simulink model "QD2_MissionCtrl_Dual_MPC"  (R2022b)
settings: Solver=ode2  StartTime=0.0  StopTime=inf  FixedStep=0.001  RelTol=1e-3  EnableMultiTasking=on
PreLoadFcn:
  | % Rutas: simulink_qdrone2 (qd2_cargar_config), lib (qd2_*.m) y la carpeta
  | % del modelo (QD2_Mission_Lib.slx de la misma versión de MATLAB).
  | qd2_d = fileparts(get_param(bdroot, 'FileName')); qd2_r = qd2_d;
  | while ~isempty(qd2_r) && ~exist(fullfile(qd2_r, 'qd2_cargar_config.m'), 'file')
  |     qd2_p = fileparts(qd2_r); if strcmp(qd2_p, qd2_r), qd2_r = ''; else, qd2_r = qd2_p; end
  | end
  | if ~isempty(qd2_r), addpath(fullfile(qd2_r, 'lib')); addpath(qd2_r); end
  | if exist(fullfile(qd2_d, 'QD2_Mission_Lib.slx'), 'file'), addpath(qd2_d); end
  | clear qd2_d qd2_r qd2_p
PostLoadFcn:
  | try, qd2_cargar_config(); catch qd2_e, warning(qd2_e.message); end
InitFcn:
  | qd2_cargar_config(bdroot);
undefined symbols (not defined in the file): _MissionCtrl, _MissionDual, datetime, Host, localhost, log_, m, qc_get_step_size, QD2CFG, QD2P, saved_data
libraries: quarc_library x43, QD2_Mission_Lib x12, simulink x11
(part 1 of 2)
Description:
  | Modelo de tierra para 2 QDrone 2 (versión MPC). Copia extendida de QD2_MissionCtrl_NoJoystick_2021a del Equipo2, generada por simulink_qdrone2/construir_modelos.m. Contrato: docs/ARQUITECTURA.md.
settings Model: SimulationMode=external  ExtModeTrigDuration=10000  Creator=Admin  LastModifiedBy=ezequ
settings SolverCC: AlgebraicLoopSolver=TrustRegion  PositivePriorityOrder=on
settings DataIOCC: ReturnWorkspaceOutputs=off
settings OptimizationCC: ReuseModelBlockBuffer=on
settings DebuggingCC: UnconnectedInputMsg=warning  UnconnectedOutputMsg=warning  UnconnectedLineMsg=warning  SFUnexpectedBacktrackingDiag=warning  SFNoUnconditionalDefaultTransitionDiag=warning  SFExecutionAtInitializationDiag=none  ArithmeticOperatorsInVariantConditions=warning
settings ModelReferenceCC: EnableRefExpFcnMdlSchedulingChecks=on
settings SFSimCC: SimUseLocalCustomCode=off  CustomCodeUndefinedFunction=UseInterfaceOnly
settings RTWCC: Description=QUARC Win64 Target Using Toolchain  SystemTargetFile=quarc_win64.tlc  TemplateMakefile=quarc_default_tmf  RTWUseLocalCustomCode=off  Toolchain=QUARC win64 | nmake (64-bit Windows)  BuildConfiguration=Faster Runs  DLArmComputeVersion=19.05
settings CodeAppCC: StateflowObjectComments=on
settings STFCustomTargetCC: ConcurrentExecutionCompliant=on  GRTInterface=on  UseToolchainInfoCompliant=on  SystemTargetFile=quarc_win64.tlc
settings GRTTargetCC: TargetLangStandard=C89/C90 (ANSI)  ParMdlRefBuildCompliant=off  CompOptLevelCompliant=off  CombineOutputUpdateFcns=off  MatFileLogging=off  CPPClassGenCompliant=off  GRTInterface=on  ExtMode=on  ExtModeMexFile=quarc_comm  ExtModeMexArgs='-w -d %d -uri %u -URI_Host tcpip://localhost:18001 -URI_Host2 tcpip://localhost:18002'
settings ConfigComp: CovMetricSettings=dw  CovSaveCumulativeToWorkspaceVar=on  CovSaveSingleToWorkspaceVar=on  CovExternalEMLEnable=off  CovBoundaryAbsTol=1.0e-5

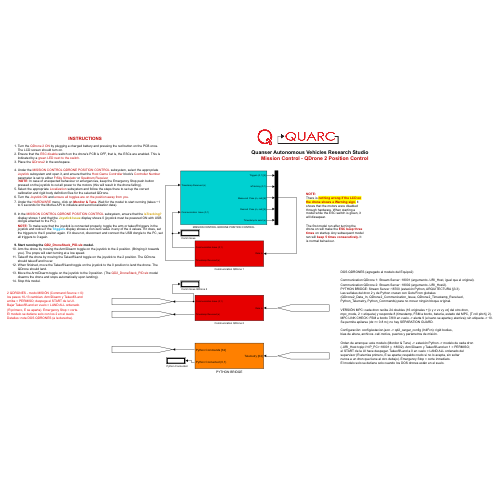
[thumbnail: Simulink's stored preview of the top-level diagram]
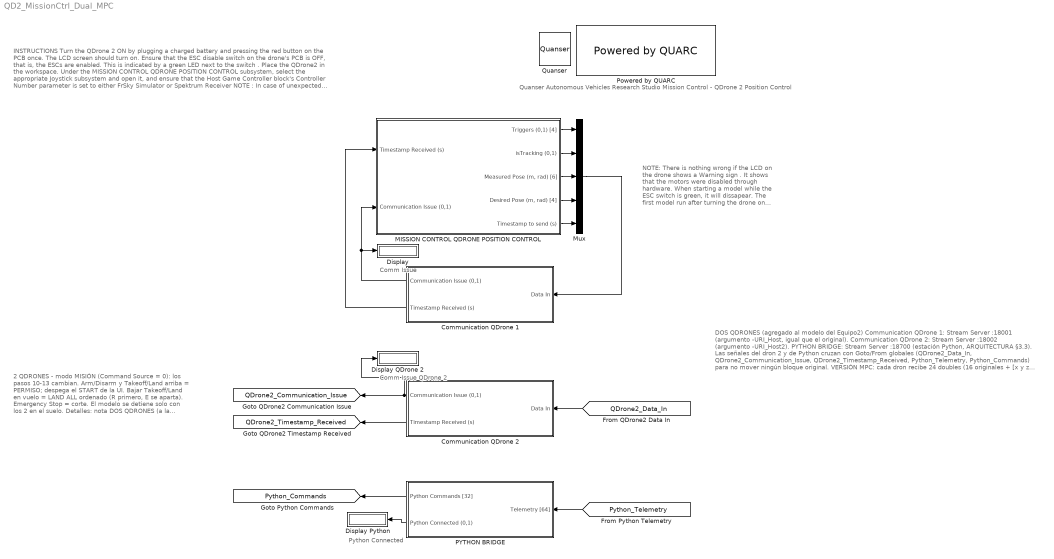
== system QD2_MissionCtrl_Dual_MPC ==
  note: Quanser Autonomous Vehicles Research Studio
      | Mission Control - QDrone 2 Position Control
  note: Comm Issue
  note: INSTRUCTIONS
      |
      | Turn the QDrone 2 ON by plugging a charged battery and pressing the red button on the PCB once. The LCD screen should turn on.
      | Ensure that the ESC disable switch on the drone's PCB is OFF, that is, the ESCs are enabled. This is indicated by a green LED next to the switch .
      | Place the QDrone2 in the workspace.
      |
      | Under the MISSION CONTROL QDRONE POSITION CONTROL subsystem, select the appropriate Joystick subsystem and open it, and ensure that the Host Game Controller block's Controller Number parameter is set to either FrSky Simulator or Spektrum Receiver
      | NOTE : In case of unexpected behaviour or emergencies, keep the Emergency Stop push button pressed on the joystick to cut all power to the motors (this will result in the drone falling).
      | Select the appropriate Localization subsystem and follow the steps there to set up the correct calibration and rigid body definition files for the selected QDrone.
      | Turn the Joystick ON and ensure all toggles are on the position away from you .
      | Under the HARDWARE menu, click on Monitor & Tune . Wait for the model to start running (takes ~1 to 5 seconds for the Motive API to initialize and send localization data).
      |
      | In the MISSION CONTROL QDRONE POSITION CONTROL subsystem, ensure that the isTracking? display shows 1 and that the Joystick Issue display shows 0 (joystick must be powered ON with USB dongle attached to the PC).
      | NOTE: To make sure that the joystick is connected properly, toggle the arm or takeoff triggers in the joystick and notice if the Triggers display shows a non zero value in any of the 4 values. If it does, set the triggers to the 0 positon again. If it does not, disconnect and connect the USB dongle to the PC, set all triggers to 0 again.
      |
      | Start running the QD2_DroneStack_PID.slx model.
      | Arm the drone by moving the Arm/Disarm toggle on the joystick to the 2 position. (Bringing it towards you). The props will start turning at a low speed.
      | Takeoff the drone by moving the Takeoff/Land toggle on the joystick to the 2 position. The QDrone should takeoff and hover.
      | When finished, move the Takeoff/Land toggle on the joystick to the 0 position to land the drone. The QDrone should land.
      | Move the Arm/Disarm toggle on the joystick to the 0 position. (The QD2_DroneStack_PID.sl x model disarms the drone and stops automatically upon landing).
      | Stop this model.
  note: NOTE:
      | There is nothing wrong if the LCD on the drone shows a Warning sign . It shows that the motors were disabled through hardware. When starting a model while the ESC switch is green, it will dissapear.
      |
      | The first model run after turning the drone on will make the ESC beep three times on startup. Any subsequent model ran will beep 5 times consecutively. It is normal behaviour.
  note: Comm Issue QDrone 2
  note: Python Connected
  note: DOS QDRONES (agregado al modelo del Equipo2)
      |
      | Communication QDrone 1: Stream Server :18001 (argumento -URI_Host, igual que el original).
      | Communication QDrone 2: Stream Server :18002 (argumento -URI_Host2).
      | PYTHON BRIDGE: Stream Server :18700 (estación Python, ARQUITECTURA §3.3).
      | Las señales del dron 2 y de Python cruzan con Goto/From globales
      | (QDrone2_Data_In, QDrone2_Communication_Issue, QDrone2_Timestamp_Received,
      | Python_Telemetry, Python_Commands) para no mover ningún bloque original.
      |
      | VERSIÓN MPC: cada dron recibe 24 doubles (16 originales + [x y z vx vy vz] del otro dron,
      | mpc_mode, 2 = etiqueta) y responde 8 (timestamp, FSM a bordo, batería, estado del MPC, [T roll pitch], 2).
      | MPC LINK CHECK: FSM a bordo 7/8/9 en vuelo -> alerta 9 (el sano se aparta y aterriza); sin etiqueta -> 10.
      | Se permite apilarse (dz >= 0.8 m); no hay SEPARATION GUARD.
      |
      | Configuración: config/estacion.json -> qd2_cargar_config (InitFcn): rigid bodies,
      | bias de altura, archivos .cal/.motive, puertos y parámetros de misión.
      |
      | Orden de arranque: este modelo (Monitor & Tune) -> estación Python -> modelo de cada dron
      | (-URI_Host tcpip://<IP_PC>:18001 y :18002). Arm/Disarm y Takeoff/Land en 1 = PERMISO;
      | el START de la UI hace despegar. Takeoff/Land a 0 en vuelo = LAND ALL ordenado del
      | supervisor (R aterriza primero, E se aparta; respaldo crudo si no lo acepta, sin soltar
      | nunca a un dron que tiene al otro debajo). Emergency Stop = corte inmediato.
      | El modelo solo se detiene solo cuando los DOS drones están en el suelo.
  note: 2 QDRONES - modo MISIÓN (Command Source = 0):
      | los pasos 10-13 cambian. Arm/Disarm y Takeoff/Land
      | arriba = PERMISO; despega el START de la UI.
      | Bajar Takeoff/Land en vuelo = LAND ALL ordenado
      | (R primero, E se aparta). Emergency Stop = corte.
      | El modelo se detiene solo con los 2 en el suelo.
      | Detalles: nota DOS QDRONES (a la derecha).
  Communication QDrone 1 : Subsystem
  Communication QDrone 2 : Subsystem
  Display : Display
  Display Python : Display
  Display QDrone 2 : Display
  MISSION CONTROL QDRONE POSITION CONTROL : Subsystem
  Mux : Mux  Inputs=5
  PYTHON BRIDGE : Subsystem
  Powered by QUARC : quarc_library/Logos/Powered by QUARC
  Quanser : quarc_library/Logos/Quanser
  tag scope: Python_Commands=global, QDrone2_Communication_Issue=global, QDrone2_Timestamp_Received=global
  wires:
  Communication QDrone 1/2(Timestamp Received (s)) -> MISSION CONTROL QDRONE POSITION CONTROL/1(Timestamp Received (s))
  MISSION CONTROL QDRONE POSITION CONTROL/5(Timestamp to send (s)) -> Mux/5
  Mux/1 -> Communication QDrone 1/1(Data In)
  Communication QDrone 1/1(Communication Issue (0,1)) -> MISSION CONTROL QDRONE POSITION CONTROL/2(Communication Issue (0,1)), Display/1
  MISSION CONTROL QDRONE POSITION CONTROL/3("Measured Pose (m, rad) [6]") -> Mux/3
  MISSION CONTROL QDRONE POSITION CONTROL/4("Desired Pose (m, rad) [4]") -> Mux/4
  MISSION CONTROL QDRONE POSITION CONTROL/1(Triggers (0,1) [4]) -> Mux/1
  MISSION CONTROL QDRONE POSITION CONTROL/2(isTracking (0,1)) -> Mux/2
  [QDrone2_Data_In] -> Communication QDrone 2/1(Data In)
  Communication QDrone 2/1(Communication Issue (0,1)) -> [QDrone2_Communication_Issue], Display QDrone 2/1
  Communication QDrone 2/2(Timestamp Received (s)) -> [QDrone2_Timestamp_Received]
  [Python_Telemetry] -> PYTHON BRIDGE/1(Telemetry [64])
  PYTHON BRIDGE/1(Python Commands [32]) -> [Python_Commands]
  PYTHON BRIDGE/2(Python Connected (0,1)) -> Display Python/1

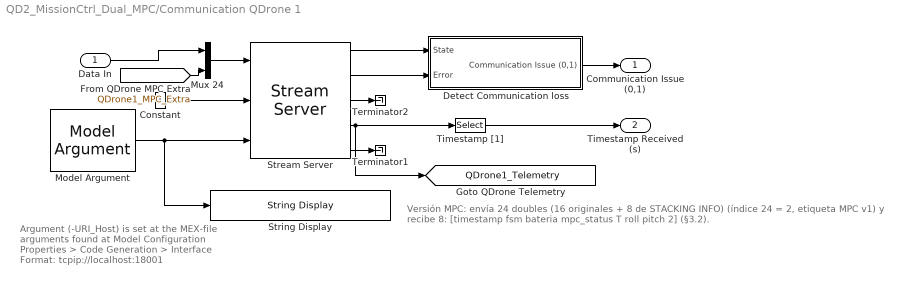
== system QD2_MissionCtrl_Dual_MPC/Communication QDrone 1 ==
  note: Argument (-URI_Host) is set at the MEX-file arguments
      | found at Model Configuration Properties > Code Generation > Interface
      |
      | Format:
      | tcpip://localhost:18001
  note: Versión MPC: envía 24 doubles (16 originales + 8 de STACKING INFO)
      | (índice 24 = 2, etiqueta MPC v1) y recibe 8: [timestamp fsm bateria mpc_status T roll pitch 2] (§3.2).
  Data In : Inport
  Constant : Constant
  Detect Communication loss : Subsystem
  Model Argument : quarc_library/Sources/Signals/Model Argument  argument_name=URI_Host  has_value=on  data_type_mode=Specify via dialog  data_type=char  max_length=80  default_value=0  variable_size=off
      settings: AttributesFormatString=(-%<argument_name>)  SourceProductName=QUARC Targets
  Mux 24 : Mux  Inputs=2
  Stream Server : quarc_library/Communications/Basic/Stream Server  uri_source=External input port  uri=tcpip://localhost:18877  send_buffer_size=1460  receive_buffer_size=1460  byte_order=little endian (Intel - LSB first)  optimization=Minimum latency  send_options=Send most recent data  receive_options=Receive most recent data  default_value=[0; NaN(7,1)]  sample_time=qc_get_step_size  active=off  implementation=Use blocking I/O in a separate thread  send_fifo_size=1000  receive_fifo_size=1000  send_priority=0  receive_priority=0  send_dimensions=off  receive_dimensions=off  max_dimensions=-1  data_type=Inherited via back propagation  type_expr=BusObject
  "String Display " : quarc_library/Strings/String Display  alignment=center  display_mode=Single line  sample_time=-1  use_new=off
      settings: SourceProductName=QUARC Targets
  Terminator1 : Terminator
  Terminator2 : Terminator
  Timestamp [1] : Selector  InputPortWidth=8  IndexOptions=Index vector (dialog)  Indices=1  OutputSizes=1
  Communication Issue (0,1) : Outport  VectorParamsAs1DForOutWhenUnconnected=off
  Timestamp Received (s) : Outport  Port=2  VectorParamsAs1DForOutWhenUnconnected=off
  tag scope: QDrone1_Telemetry=global
  wires:
  Constant/1 -> Stream Server/2
  Stream Server/3 -> Terminator2/1
  Stream Server/5 -> Terminator1/1
  Model Argument/1 -> "String Display "/1, Stream Server/3
  Stream Server/1 -> Detect Communication loss/1(State)
  Stream Server/2 -> Detect Communication loss/2(Error)
  Detect Communication loss/1(Communication Issue (0,1)) -> Communication Issue (0,1)/1
  Data In/1 -> Mux 24/1
  [QDrone1_MPC_Extra] -> Mux 24/2
  Mux 24/1 -> Stream Server/1
  Stream Server/4 -> Timestamp [1]/1, [QDrone1_Telemetry]
  Timestamp [1]/1 -> Timestamp Received (s)/1

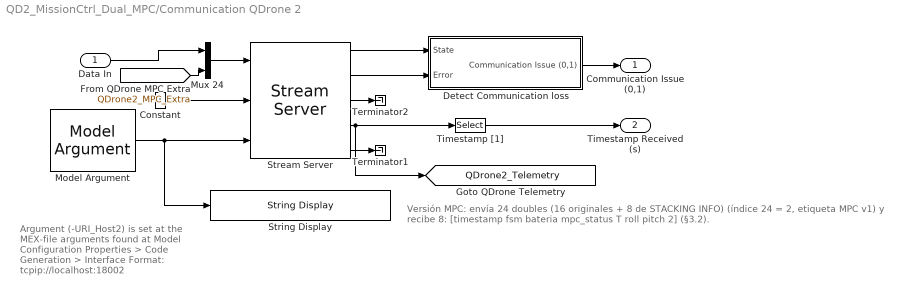
== system QD2_MissionCtrl_Dual_MPC/Communication QDrone 2 ==
  note: Versión MPC: envía 24 doubles (16 originales + 8 de STACKING INFO)
      | (índice 24 = 2, etiqueta MPC v1) y recibe 8: [timestamp fsm bateria mpc_status T roll pitch 2] (§3.2).
  note: Argument (-URI_Host2) is set at the MEX-file arguments
      | found at Model Configuration Properties > Code Generation > Interface
      |
      | Format:
      | tcpip://localhost:18002
  Data In : Inport
  Constant : Constant
  Detect Communication loss : Subsystem
  Model Argument : quarc_library/Sources/Signals/Model Argument  argument_name=URI_Host2  has_value=on  data_type_mode=Specify via dialog  data_type=char  max_length=80  default_value=0  variable_size=off
      settings: AttributesFormatString=(-%<argument_name>)  SourceProductName=QUARC Targets
  Mux 24 : Mux  Inputs=2
  Stream Server : quarc_library/Communications/Basic/Stream Server  uri_source=External input port  uri=tcpip://localhost:18877  send_buffer_size=1460  receive_buffer_size=1460  byte_order=little endian (Intel - LSB first)  optimization=Minimum latency  send_options=Send most recent data  receive_options=Receive most recent data  default_value=[0; NaN(7,1)]  sample_time=qc_get_step_size  active=off  implementation=Use blocking I/O in a separate thread  send_fifo_size=1000  receive_fifo_size=1000  send_priority=0  receive_priority=0  send_dimensions=off  receive_dimensions=off  max_dimensions=-1  data_type=Inherited via back propagation  type_expr=BusObject
  "String Display " : quarc_library/Strings/String Display  alignment=center  display_mode=Single line  sample_time=-1  use_new=off
      settings: SourceProductName=QUARC Targets
  Terminator1 : Terminator
  Terminator2 : Terminator
  Timestamp [1] : Selector  InputPortWidth=8  IndexOptions=Index vector (dialog)  Indices=1  OutputSizes=1
  Communication Issue (0,1) : Outport  VectorParamsAs1DForOutWhenUnconnected=off
  Timestamp Received (s) : Outport  Port=2  VectorParamsAs1DForOutWhenUnconnected=off
  tag scope: QDrone2_Telemetry=global
  wires:
  Timestamp [1]/1 -> Timestamp Received (s)/1
  Stream Server/4 -> [QDrone2_Telemetry], Timestamp [1]/1
  Mux 24/1 -> Stream Server/1
  [QDrone2_MPC_Extra] -> Mux 24/2
  Data In/1 -> Mux 24/1
  Detect Communication loss/1(Communication Issue (0,1)) -> Communication Issue (0,1)/1
  Stream Server/2 -> Detect Communication loss/2(Error)
  Stream Server/1 -> Detect Communication loss/1(State)
  Model Argument/1 -> Stream Server/3, "String Display "/1
  Stream Server/5 -> Terminator1/1
  Stream Server/3 -> Terminator2/1
  Constant/1 -> Stream Server/2

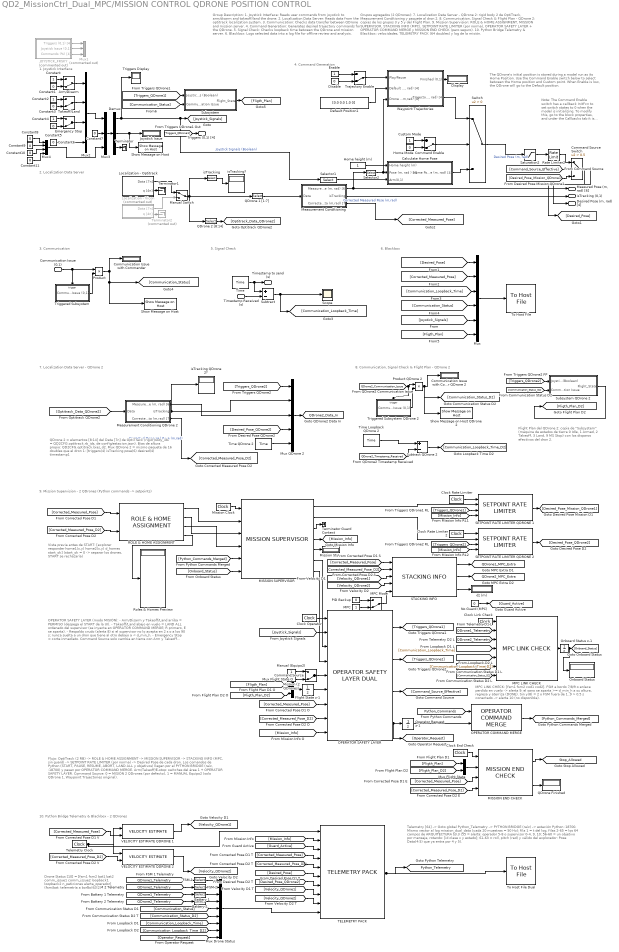
== system QD2_MissionCtrl_Dual_MPC/MISSION CONTROL QDRONE POSITION CONTROL ==
  note: 5. Signal Check
  note: 6. Blackbox
  note: 3. Communication
  note: 2. Localization Data Server
  note: 1. Joystick Interface
  note: 4. Command Generation
  note: Group Description:
      |
      | 1. Joystick Interface: Reads user commands from joystick to arm/disarm and takeoff/land the drone.
      | 2. Localization Data Server: Reads data from the optitrack localization system.
      | 3. Communication: Checks data transfer between QDrone and mission server.
      | 4. Command Generation: Generates desired trajectory commands for the QDrone.
      | 5. Signal Check: Checks loopback time between the QDrone and mission server.
      | 6. Blackbox: Logs selected data into a log file for offline review and analysis.
  note: The QDrone's initial position is stored during a model run as its Home Position.
      | Use the Command Enable switch below to select between the Home position and Custom point. When Enable is low, the QDrone will go to the Default position.
  note: Note:
      | The Command Enable switch has a callback InitFcn to set switch states to 0 when the model is initializing. To modify this, go to the block properties, and under the Callbacks tab it is set in the InitFcn.
  note: 7. Localization Data Server - QDrone 2
  note: 8. Communication, Signal Check & Flight Plan - QDrone 2
  note: 9. Mission Supervision - 2 QDrones (Python commands -> setpoints)
  note: 10. Python Bridge Telemetry & Blackbox - 2 QDrones
  note: Grupos agregados (2 QDrones):
      |
      | 7. Localization Data Server - QDrone 2: rigid body 2 de OptiTrack, Measurement Conditioning y paquete al dron 2.
      | 8. Communication, Signal Check & Flight Plan - QDrone 2: copias de los grupos 3 y 5 y del Flight Plan.
      | 9. Mission Supervision: ROLE & HOME ASSIGNMENT, MISSION SUPERVISOR, STACKING INFO (MPC),
      |    SETPOINT RATE LIMITER (por norma), OPERATOR SAFETY LAYER + OPERATOR COMMAND MERGE y MISSION END CHECK (paro seguro).
      | 10. Python Bridge Telemetry & Blackbox: velocidades, TELEMETRY PACK (64 doubles) y log de la misión.
  note: QDrone 2 = elementos [8:14] del Data [7n] de OptiTrack
      | (rigid_body_ids = QD2CFG.optitrack.rb_ids, de config/estacion.json).
      | Bias de altura propio: QD2CFG.optitrack.bias_d2.
      | Mux QDrone 2 = mismo paquete de 16 doubles que el dron 1:
      | [triggers(4) isTracking pose(6) desired(4) timestamp].
  note: Flight Plan del QDrone 2: copia de "Subsystem"
      | (máquina de estados de tierra 0 Idle, 1 Armed,
      | 2 Takeoff, 3 Land, 9 MS Stop) con los disparos
      | efectivos del dron 2.
  note: Vista previa antes de START:
      | [explorer responder home1(x,y) home2(x,y)
      |  d_homes start_ok]  (start_ok = 0 ->
      |  separar los drones, START se rechazaría)
  note: OPERATOR SAFETY LAYER (modo MISIÓN):
      | - Arm/Disarm y Takeoff/Land arriba = PERMISO (despega el START de la UI).
      | - Takeoff/Land abajo en vuelo = LAND ALL ordenado del supervisor
      |   (se inyecta en OPERATOR COMMAND MERGE; R primero, E se aparta).
      | - Respaldo crudo (alerta 8) si el supervisor no lo acepta en 2 s o a los
      |   90 s; nunca suelta a un dron que tiene al otro debajo a < d_min_h.
      | - Emergency Stop = corte inmediato. Command Source solo cambia en
      |   tierra con Arm y Takeoff abajo.
  note: MPC LINK CHECK: [fsm1 fsm2 cod1 cod2]. FSM a bordo 7/8/9 o enlace perdido en vuelo
      | -> alerta 9: el sano se aparta >= d_min_h a su altura, regresa y aterriza (DONE).
      | Sin y(8) = 2 o FSM fuera de 1..9 > 0.5 s conectado -> alerta 10 (no disponible).
  note: Flujo: OptiTrack (2 RB) -> ROLE & HOME ASSIGNMENT -> MISSION SUPERVISOR -> STACKING INFO (MPC, sin guard)
      | -> SETPOINT RATE LIMITER (por norma) -> Desired Pose de cada dron. Los comandos de Python (START, PAUSE, RESUME,
      | ABORT, LAND ALL y objetivos) llegan por el PYTHON BRIDGE (raíz, :18700) y pasan por OPERATOR COMMAND MERGE.
      | Arm/Takeoff/E-stop: switches del área 1 + OPERATOR SAFETY LAYER. Command Source: 0 = MISIÓN 2 QDrones (por defecto),
      | 1 = MANUAL Equipo2 (solo QDrone 1, Waypoint Trajectories original).
  note: Drone Status [10] = [fsm1 fsm2 bat1 bat2
      | comm_issue1 comm_issue2 loopback1
      | loopback2 n_peticiones alerta_operador]
      | (fsm/bat: telemetría a bordo, §3.2)
  note: Telemetry [64] -> Goto global Python_Telemetry -> PYTHON BRIDGE (raíz) -> estación Python :18700.
      | Mismo vector al log mission_dual_data (cada 20 muestras = 50 Hz): fila 1 = t del log,
      | filas 2-65 = los 64 campos de ARQUITECTURA §3.3 (55 = alerta: operador 5-8 o supervisor 0-4, 9, 10;
      | 56-60 = un objetivo por mensaje, rotando: [id clase x y estado];
      | 61-63 = roll, pitch (rad) y válido del explorador: Pose Data(4:5) que ya entra por 4 y 5).
  Timestamp Received (s) : Inport
  Communication Issue (0,1) : Inport  Port=2
  Arm/Disarm : ManualSwitch  InitFcn=set_param(gcb,'sw','0')  CurrentSetting=0
  Battery 1 : Selector  InputPortWidth=8  IndexOptions=Index vector (dialog)  Indices=3  OutputSizes=1
  Battery 2 : Selector  InputPortWidth=8  IndexOptions=Index vector (dialog)  Indices=3  OutputSizes=1
  Calculate Home Pose : Subsystem
  Clock End Check : DigitalClock  SampleTime=qc_get_step_size
  Clock Link Check : DigitalClock  SampleTime=qc_get_step_size
  Clock Operator : DigitalClock  SampleTime=qc_get_step_size
  Clock Rate Limiter : DigitalClock  SampleTime=qc_get_step_size
  Clock Rate Limiter 2 : DigitalClock  SampleTime=qc_get_step_size
  Command Enable : ManualSwitch  InitFcn=set_param(gcb,'sw','0')  CurrentSetting=0
  Command Source : ManualSwitch  InitFcn=set_param(gcb,'sw','0')  CurrentSetting=0
  Command Source Switch : Switch  Criteria=u2 > Threshold  Threshold=0.5  SaturateOnIntegerOverflow=off  InputSameDT=off
  Communication Issue with Commander : Display
  Communication Issue with Commander QDrone 2 : Display
  Constant : Constant
  Constant{1,3,5..11} (9 alike) : Constant  Value=0
  Constant2 : Constant
  Constant4 : Constant
  Custom Mode : Constant
  Default Position1 : Constant  Value=[0.0 0.0 1.0 0]
  Demux : Demux  Outputs=[4 1 4]
  Disable : Constant  Value=0
  Display : Display
  Emergency Stop : ManualSwitch  InitFcn=set_param(gcb,'sw','0')  CurrentSetting=0
  Enable : Constant
  FSM 1 : Selector  InputPortWidth=8  IndexOptions=Index vector (dialog)  Indices=2  OutputSizes=1
  FSM 2 : Selector  InputPortWidth=8  IndexOptions=Index vector (dialog)  Indices=2  OutputSizes=1
  Flight State z-1 : UnitDelay  InitialCondition=[0; 0]  SampleTime=qc_get_step_size  HasFrameUpgradeWarning=on
  Home Mode : Constant  Value=0
  Home height (m) : Constant
  JOYSTICK_FRSKY : Subsystem  Commented=on
      mask Display: image('$imagefile'); % Use "Edit Image" on toolstrip to change.
  Joystick Issue : Display
  Localization - Optitrack : Subsystem
      mask Display: image('$imagefile'); % Use "Edit Image" on toolstrip to change.
  Localization - Vicon : Subsystem  Commented=on
      mask Display: image('$imagefile'); % Use "Edit Image" on toolstrip to change.
  MISSION END CHECK : QD2_Mission_Lib/MISSION END CHECK  Ts=qc_get_step_size
  MISSION SUPERVISOR : QD2_Mission_Lib/MISSION SUPERVISOR  P=QD2P  version=2  Ts=qc_get_step_size
  MPC : Constant
  MPC LINK CHECK : QD2_Mission_Lib/MPC LINK CHECK  P=QD2P  version=2  Ts=qc_get_step_size
  MPC Mode : ManualSwitch  InitFcn=set_param(gcb,'sw','0')  CurrentSetting=0
  Manual (Equipo2) : Constant
  Manual Switch : ManualSwitch
  Measurement Conditioning : Subsystem
  Measurement Conditioning QDrone 2 : Subsystem
  Mission (2 QDrones) : Constant  Value=0
  Mission Clock : DigitalClock  SampleTime=qc_get_step_size
  Mission State : Display
  Mux : Mux  Inputs=6
  Mux Drone Status : Mux  Inputs=[1 1 1 1 1 1 1 1 2]
  Mux Flight State : Mux  Inputs=2
  Mux Flight State O : Mux  Inputs=2
  Mux QDrone 2 : Mux  Inputs=5
  Mux1 : Mux  Commented=on  Inputs=[4 1 4]
  Mux2 : Mux
  Mux3 : Mux  Inputs=3
  Mux4 : Mux
  No Guard (MPC) : Constant  Value=0
  OPERATOR COMMAND MERGE : QD2_Mission_Lib/OPERATOR COMMAND MERGE  Ts=qc_get_step_size
  OPERATOR SAFETY LAYER : QD2_Mission_Lib/OPERATOR SAFETY LAYER DUAL  P=QD2P  Ts=qc_get_step_size
  Onboard Status : Display
  Onboard Status z-1 : UnitDelay  InitialCondition=[0; 0; 0; 0]  SampleTime=qc_get_step_size  HasFrameUpgradeWarning=on
  Operator Request z-1 : UnitDelay  InitialCondition=[0; 0]  SampleTime=qc_get_step_size  HasFrameUpgradeWarning=on
  PID Backup : Constant  Value=0
  Product : Product
  Product QDrone 2 : Product
  QDrone 1 [1:7] : Selector  InputPortWidth=14  IndexOptions=Index vector (dialog)  Indices=1:7  OutputSizes=1
  QDrone 2 [8:14] : Selector  InputPortWidth=14  IndexOptions=Index vector (dialog)  Indices=8:14  OutputSizes=1
  QDrone Finished : Display
  ROLE & HOME ASSIGNMENT : QD2_Mission_Lib/ROLE & HOME ASSIGNMENT  P=QD2P  version=2  Ts=qc_get_step_size
  Rate Limiter2 : RateLimiter  RisingSlewLimit=[1/3 1/3 1/6 pi/6]  FallingSlewLimit=[-1/3 -1/3 -1/6 -pi/6]  SampleTimeMode=inherited
  Roles & Homes Preview : Display
  SETPOINT RATE LIMITER QDRONE 1 : QD2_Mission_Lib/SETPOINT RATE LIMITER  P=QD2P  dron=1  Ts=qc_get_step_size
  SETPOINT RATE LIMITER QDRONE 2 : QD2_Mission_Lib/SETPOINT RATE LIMITER  P=QD2P  dron=2  Ts=qc_get_step_size
  STACKING INFO : QD2_Mission_Lib/STACKING INFO  Ts=qc_get_step_size
  Saturation2 : Saturate  UpperLimit=[1.5 1.5 1.5 3*pi]  LowerLimit=[-1.5 -1.5 0 -3*pi]
  Scope : Scope
  Selector1 : Selector  InputPortWidth=4  IndexOptions=Index vector (dialog)  Indices=[1]  OutputSizes=1
  Selector2 : Selector  InputPortWidth=6  IndexOptions=Index vector (dialog)  Indices=[1:3,6]  OutputSizes=1
  Show Message on Host : quarc_library/Sinks/Error Handling/Show Message on Host  message_type=Fixed error message  message_icon=Warning  message=Mission Control: No communication with QDrone
      settings: AttributesFormatString="\"%<message>\""  SourceProductName=QUARC Targets
  "Show Message on Host " : quarc_library/Sinks/Error Handling/Show Message on Host  message_type=Fixed error message  message_icon=Warning  message=Mission Control: Joystick Disconnected
      settings: AttributesFormatString="\"%<message>\""  SourceProductName=QUARC Targets
  Show Message on Host QDrone 2 : quarc_library/Sinks/Error Handling/Show Message on Host  message_type=Fixed error message  message_icon=Warning  message=Mission Control: No communication with QDrone 2
      settings: AttributesFormatString="\"%<message>\""  SourceProductName=QUARC Targets
  Subsystem : Subsystem
  Subsystem QDrone 2 : Subsystem
  Subtract : Sum  Inputs=+-
  Subtract QDrone 2 : Sum  Inputs=+-
  Switch : Switch  Criteria=u2 > Threshold  SaturateOnIntegerOverflow=off  InputSameDT=off
  TELEMETRY PACK : QD2_Mission_Lib/TELEMETRY PACK  version=2  Ts=qc_get_step_size
  Takeoff/Land : ManualSwitch  InitFcn=set_param(gcb,'sw','0')  CurrentSetting=0
  Telemetry Clock : DigitalClock  SampleTime=qc_get_step_size
  Terminator : Terminator
  Terminator Guard Context : Terminator
  Terminator1 : Terminator
  Terminator2 : Terminator  Commented=on
  Time : quarc_library/Sources/Time/Time  time_source=Wall clock  sample_time=qc_get_step_size
  Time Loopback QDrone 2 : quarc_library/Sources/Time/Time  time_source=Wall clock  sample_time=qc_get_step_size
  Time QDrone 2 : quarc_library/Sources/Time/Time  time_source=Wall clock  sample_time=qc_get_step_size
  To Host File : quarc_library/Sinks/To Host/To Host File  source=Specify via dialog (do not evaluate)  file_name=saved_data/%m/log_%{regexprep(char(datetime),' ','_')}_MissionCtrl.mat  variable_name=mission_server_data  decimation=1  sample_time=-1  file_format=MAT-file v.5  options=No header or footer  append=off  final_file_name=saved_data/QD2_MissionCtrl_Dual_MPC/log_22-Nov-2026_19-01-13_MissionCtrl.mat  encoding=Default  bitrate=2000000
  To Host File Dual : quarc_library/Sinks/To Host/To Host File  source=Specify via dialog (do not evaluate)  file_name=saved_data/%m/log_%{regexprep(char(datetime),' ','_')}_MissionDual.mat  variable_name=mission_dual_data  decimation=20  sample_time=-1  file_format=MAT-file v.5  options=No header or footer  append=off  final_file_name=saved_data/QD2_MissionCtrl_Dual_MPC/log_22-Nov-2026_19-01-13_MissionDual.mat  encoding=Default  bitrate=2000000
  Trajectory Enable : ManualSwitch  InitFcn=set_param(gcb,'sw','0')  CurrentSetting=0
  Triggered Subsystem : Subsystem  TreatAsAtomicUnit=on
  Triggered Subsystem QDrone 2 : Subsystem  TreatAsAtomicUnit=on
  Triggers Display : Display
  VELOCITY ESTIMATE QDRONE 1 : QD2_Mission_Lib/VELOCITY ESTIMATE  Ts=qc_get_step_size
  VELOCITY ESTIMATE QDRONE 2 : QD2_Mission_Lib/VELOCITY ESTIMATE  Ts=qc_get_step_size
  Waypoint Trajectories : Subsystem
  dz (m) : Display
  isTracking : Selector  InputPortWidth=14  IndexOptions=Index vector (dialog)  Indices=[7]  OutputSizes=1
  isTracking QDrone 2? : Display
  isTracking? : Display
  Triggers (0,1) [4] : Outport  VectorParamsAs1DForOutWhenUnconnected=off
  isTracking (0,1) : Outport  Port=2  VectorParamsAs1DForOutWhenUnconnected=off
  "Measured Pose (m, rad) [6]" : Outport  Port=3  VectorParamsAs1DForOutWhenUnconnected=off
  "Desired Pose (m, rad) [4]" : Outport  Port=4  VectorParamsAs1DForOutWhenUnconnected=off
  Timestamp to send (s) : Outport  Port=5  VectorParamsAs1DForOutWhenUnconnected=off
  tag scope: Python_Telemetry=global, QDrone1_MPC_Extra=global, QDrone2_Data_In=global, QDrone2_MPC_Extra=global, Stop_Allowed=global
  wires:
  Communication Issue (0,1)/1 -> Product/1, Triggered Subsystem/Trigger
  isTracking/1 -> isTracking?/1
  Demux/2 -> "Show Message on Host "/1, Joystick Issue/1
  Demux/3 -> Terminator/1
  Demux/1 -> [Joystick_Signals], Selector1/1, Triggers Display/1  "Joystick Signals (Boolean)"
  Time/1 -> Subtract/1, Timestamp to send (s)/1
  Timestamp Received (s)/1 -> Subtract/2
  Subtract/1 -> Scope/1, [Communication_Loopback_Time]
  Switch/1 -> Saturation2/1  "Desired Pose (m, rad)"
  Measurement Conditioning/2(isTracking) -> isTracking (0,1)/1
  Home height (m)/1 -> Calculate Home Pose/1(Home height (m))
  Triggered Subsystem/1(Communication Issue (0,1)) -> Product/2
  Mux/1 -> To Host File/1
  Selector1/1 -> Calculate Home Pose/3(Arm(0,1))
  Measurement Conditioning/1("Measured Pose (m, rad) [6]") -> "Measured Pose (m, rad) [6]"/1, Selector2/1
  Measurement Conditioning/3(Corrected Pose Data (m,rad) [7]) -> [Corrected_Measured_Pose]  "Corrected Measured Pose (m,rad)"
  Localization - Optitrack/1(Data [7n]) -> Manual Switch/1
  Localization - Vicon/1(Data [7n]) -> Manual Switch/2
  Constant/1 -> Arm/Disarm/1
  Home Mode/1 -> Command Enable/2
  Custom Mode/1 -> Command Enable/1
  JOYSTICK_FRSKY/2(Joystick Issue (0,1)) -> Mux1/2
  JOYSTICK_FRSKY/1(Triggers (0,1) [4]) -> Mux1/1
  JOYSTICK_FRSKY/3(Commands (%) [4]) -> Mux1/3
  Manual Switch/1 -> isTracking/1, QDrone 1 [1:7]/1, QDrone 2 [8:14]/1
  Selector2/1 -> Waypoint Trajectories/3(Drone Pose (m,rad) [4]), Calculate Home Pose/2("Pose (m, rad ) [4]")
  Localization - Optitrack/2(q [4n]) -> Terminator1/1
  Localization - Vicon/2(q [4n]) -> Terminator2/1
  [Joystick_Signals] -> Mux/5
  [Desired_Pose] -> Mux/1
  [Corrected_Measured_Pose] -> Mux/2
  [Communication_Loopback_Time] -> Mux/3
  [Communication_Status] -> Mux/4
  Subsystem/1(Flight_State) -> [Fligth_Plan]
  [Fligth_Plan] -> Mux/6
  [Communication_Status] -> Subsystem/2("Communication Issue ")
  Product/1 -> Communication Issue with Commander/1, [Communication_Status], Show Message on Host/1
  Constant1/1 -> Arm/Disarm/2
  Constant3/1 -> Takeoff/Land/2
  Constant2/1 -> Takeoff/Land/1
  Takeoff/Land/1 -> Mux2/2
  Arm/Disarm/1 -> Mux2/1
  Emergency Stop/1 -> Mux2/3
  Constant4/1 -> Emergency Stop/1
  Constant5/1 -> Emergency Stop/2
  Constant6/1 -> Mux2/4
  Mux2/1 -> Mux3/1
  Mux3/1 -> Demux/1
  Constant7/1 -> Mux3/2
  Constant8/1 -> Mux4/1
  Constant9/1 -> Mux4/2
  Constant10/1 -> Mux4/3
  Constant11/1 -> Mux4/4
  Mux4/1 -> Mux3/3
  Saturation2/1 -> Rate Limiter2/1
  Command Enable/1 -> Switch/2
  Calculate Home Pose/1("Home Pose (m, rad) [4]") -> Switch/3
  Enable/1 -> Trajectory Enable/1
  Default Position1/1 -> Waypoint Trajectories/2("Default (m, rad) [4]")
  Trajectory Enable/1 -> Waypoint Trajectories/1(Play/Pause)
  Disable/1 -> Trajectory Enable/2
  Waypoint Trajectories/1(Finished (0,1)) -> Display/1
  Waypoint Trajectories/2("Trajectory (m, rad) [4]") -> Switch/1
  QDrone 1 [1:7]/1 -> Measurement Conditioning/1(Data)
  QDrone 2 [8:14]/1 -> [Optitrack_Data_QDrone2]
  [Triggers_QDrone1] -> Subsystem/1(Joystick Signals (Boolean))
  [Triggers_QDrone1] -> Triggers (0,1) [4]/1
  Rate Limiter2/1 -> Command Source Switch/1
  [Command_Source_Effective] -> Command Source Switch/2
  [Desired_Pose_Mission_QDrone1] -> Command Source Switch/3
  Command Source Switch/1 -> "Desired Pose (m, rad) [4]"/1, [Desired_Pose]
  [Optitrack_Data_QDrone2] -> Measurement Conditioning QDrone 2/1(Data)
  [Triggers_QDrone2] -> Mux QDrone 2/1
  Measurement Conditioning QDrone 2/2(isTracking) -> Mux QDrone 2/2, isTracking QDrone 2?/1
  Measurement Conditioning QDrone 2/1("Measured Pose (m, rad) [6]") -> Mux QDrone 2/3
  [Desired_Pose_QDrone2] -> Mux QDrone 2/4
  Time QDrone 2/1 -> Mux QDrone 2/5
  Measurement Conditioning QDrone 2/3(Corrected Pose Data (m,rad) [7]) -> [Corrected_Measured_Pose_D2]  "Corrected Measured Pose (m,rad)"
  Mux QDrone 2/1 -> [QDrone2_Data_In]
  [QDrone2_Communication_Issue] -> Product QDrone 2/1, Triggered Subsystem QDrone 2/Trigger
  Triggered Subsystem QDrone 2/1(Communication Issue (0,1)) -> Product QDrone 2/2
  Product QDrone 2/1 -> Communication Issue with Commander QDrone 2/1, [Communication_Status_D2], Show Message on Host QDrone 2/1
  Time Loopback QDrone 2/1 -> Subtract QDrone 2/1
  [QDrone2_Timestamp_Received] -> Subtract QDrone 2/2
  Subtract QDrone 2/1 -> [Communication_Loopback_Time_D2]
  [Triggers_QDrone2] -> Subsystem QDrone 2/1(Joystick Signals (Boolean))
  [Communication_Status_D2] -> Subsystem QDrone 2/2("Communication Issue ")
  Subsystem QDrone 2/1(Flight_State) -> [Fligth_Plan_D2]
  [Onboard_Status] -> MISSION SUPERVISOR/6
  [Corrected_Measured_Pose] -> ROLE & HOME ASSIGNMENT/1
  [Corrected_Measured_Pose_D2] -> ROLE & HOME ASSIGNMENT/2
  ROLE & HOME ASSIGNMENT/4 -> Roles & Homes Preview/1
  Mission Clock/1 -> MISSION SUPERVISOR/1
  ROLE & HOME ASSIGNMENT/1 -> MISSION SUPERVISOR/2
  ROLE & HOME ASSIGNMENT/2 -> MISSION SUPERVISOR/3
  ROLE & HOME ASSIGNMENT/3 -> MISSION SUPERVISOR/4
  [Python_Commands_Merged] -> MISSION SUPERVISOR/5
  MISSION SUPERVISOR/4 -> [Mission_Info]
  MISSION SUPERVISOR/5 -> Mission State/1
  PID Backup/1 -> MPC Mode/1
  MPC/1 -> MPC Mode/2
  MPC Mode/1 -> STACKING INFO/5
  [Corrected_Measured_Pose] -> STACKING INFO/1
  [Corrected_Measured_Pose_D2] -> STACKING INFO/2
  [Velocity_QDrone1] -> STACKING INFO/3
  [Velocity_QDrone2] -> STACKING INFO/4
  STACKING INFO/1 -> [QDrone1_MPC_Extra]
  STACKING INFO/2 -> [QDrone2_MPC_Extra]
  STACKING INFO/3 -> dz (m)/1
  No Guard (MPC)/1 -> [Guard_Active]
  MISSION SUPERVISOR/3 -> Terminator Guard Context/1
  Clock Rate Limiter/1 -> SETPOINT RATE LIMITER QDRONE 1/1
  [Triggers_QDrone1] -> SETPOINT RATE LIMITER QDRONE 1/3
  [Mission_Info] -> SETPOINT RATE LIMITER QDRONE 1/4
  Clock Rate Limiter 2/1 -> SETPOINT RATE LIMITER QDRONE 2/1
  [Triggers_QDrone2] -> SETPOINT RATE LIMITER QDRONE 2/3
  [Mission_Info] -> SETPOINT RATE LIMITER QDRONE 2/4
  MISSION SUPERVISOR/1 -> SETPOINT RATE LIMITER QDRONE 1/2
  MISSION SUPERVISOR/2 -> SETPOINT RATE LIMITER QDRONE 2/2
  SETPOINT RATE LIMITER QDRONE 1/1 -> [Desired_Pose_Mission_QDrone1]
  SETPOINT RATE LIMITER QDRONE 2/1 -> [Desired_Pose_QDrone2]
  Manual (Equipo2)/1 -> Command Source/1
  Mission (2 QDrones)/1 -> Command Source/2
  Clock Operator/1 -> OPERATOR SAFETY LAYER/1
  [Joystick_Signals] -> OPERATOR SAFETY LAYER/2
  MISSION SUPERVISOR/6 -> OPERATOR SAFETY LAYER/3
  MISSION SUPERVISOR/7 -> OPERATOR SAFETY LAYER/4
  Command Source/1 -> OPERATOR SAFETY LAYER/5
  [Fligth_Plan] -> Mux Flight State O/1
  [Fligth_Plan_D2] -> Mux Flight State O/2
  Mux Flight State O/1 -> Flight State z-1/1
  Flight State z-1/1 -> OPERATOR SAFETY LAYER/6
  [Corrected_Measured_Pose] -> OPERATOR SAFETY LAYER/7
  [Corrected_Measured_Pose_D2] -> OPERATOR SAFETY LAYER/8
  [Mission_Info] -> OPERATOR SAFETY LAYER/9
  OPERATOR SAFETY LAYER/1 -> [Triggers_QDrone1]
  OPERATOR SAFETY LAYER/2 -> [Triggers_QDrone2]
  OPERATOR SAFETY LAYER/3 -> [Command_Source_Effective]
  OPERATOR SAFETY LAYER/4 -> Operator Request z-1/1, [Operator_Request]
  Operator Request z-1/1 -> OPERATOR COMMAND MERGE/2
  [Python_Commands] -> OPERATOR COMMAND MERGE/1
  OPERATOR COMMAND MERGE/1 -> [Python_Commands_Merged]
  Clock Link Check/1 -> MPC LINK CHECK/1
  [QDrone1_Telemetry] -> MPC LINK CHECK/2
  [QDrone2_Telemetry] -> MPC LINK CHECK/3
  [Communication_Loopback_Time] -> MPC LINK CHECK/4
  [Communication_Loopback_Time_D2] -> MPC LINK CHECK/5
  [Communication_Status] -> MPC LINK CHECK/6
  [Communication_Status_D2] -> MPC LINK CHECK/7
  MPC LINK CHECK/1 -> Onboard Status z-1/1
  Onboard Status z-1/1 -> [Onboard_Status], Onboard Status/1
  [Fligth_Plan] -> Mux Flight State/1
  [Fligth_Plan_D2] -> Mux Flight State/2
  Clock End Check/1 -> MISSION END CHECK/1
  Mux Flight State/1 -> MISSION END CHECK/2
  [Corrected_Measured_Pose] -> MISSION END CHECK/3
  [Corrected_Measured_Pose_D2] -> MISSION END CHECK/4
  MISSION END CHECK/1 -> [Stop_Allowed]
  MISSION END CHECK/2 -> QDrone Finished/1
  Telemetry Clock/1 -> VELOCITY ESTIMATE QDRONE 1/1, VELOCITY ESTIMATE QDRONE 2/1, TELEMETRY PACK/1
  [Corrected_Measured_Pose] -> VELOCITY ESTIMATE QDRONE 1/2
  [Corrected_Measured_Pose_D2] -> VELOCITY ESTIMATE QDRONE 2/2
  VELOCITY ESTIMATE QDRONE 1/1 -> [Velocity_QDrone1]
  VELOCITY ESTIMATE QDRONE 2/1 -> [Velocity_QDrone2]
  [QDrone1_Telemetry] -> FSM 1/1
  FSM 1/1 -> Mux Drone Status/1
  [QDrone2_Telemetry] -> FSM 2/1
  FSM 2/1 -> Mux Drone Status/2
  [QDrone1_Telemetry] -> Battery 1/1
  Battery 1/1 -> Mux Drone Status/3
  [QDrone2_Telemetry] -> Battery 2/1
  Battery 2/1 -> Mux Drone Status/4
  [Communication_Status] -> Mux Drone Status/5
  [Communication_Status_D2] -> Mux Drone Status/6
  [Communication_Loopback_Time] -> Mux Drone Status/7
  [Communication_Loopback_Time_D2] -> Mux Drone Status/8
  [Operator_Request] -> Mux Drone Status/9
  [Mission_Info] -> TELEMETRY PACK/2
  [Guard_Active] -> TELEMETRY PACK/3
  [Corrected_Measured_Pose] -> TELEMETRY PACK/4
  [Corrected_Measured_Pose_D2] -> TELEMETRY PACK/5
  [Desired_Pose] -> TELEMETRY PACK/6
  [Desired_Pose_QDrone2] -> TELEMETRY PACK/7
  [Velocity_QDrone1] -> TELEMETRY PACK/8
  [Velocity_QDrone2] -> TELEMETRY PACK/9
  Mux Drone Status/1 -> TELEMETRY PACK/10
  TELEMETRY PACK/1 -> [Python_Telemetry], To Host File Dual/1

== system QD2_MissionCtrl_Dual_MPC/PYTHON BRIDGE ==
  note: PYTHON BRIDGE (ARQUITECTURA §3.3): Simulink es el Stream Server en QD2CFG.uri_puente = tcpip://localhost:18700
      | (puerto red.puerto_puente de config/estacion.json). La estación Python (web/) es el cliente TCP.
      | Envía 64 doubles de telemetría a 50 Hz y recibe 32 doubles de comandos/detecciones (most recent data).
      | Sin cliente conectado la salida queda en ceros (heartbeat = 0): el MISSION SUPERVISOR no arranca la misión
      | y, si ya estaba en MISSION, pasa a PAUSED al perder el heartbeat más de 1 s.
  Telemetry [64] : Inport
  Connected : simulink/Logic and Bit Operations/Compare To Constant  relop===  const=2  OutDataTypeStr=boolean
  Constant : Constant
  Data Type Conversion : DataTypeConversion  OutDataTypeStr=double  SaturateOnIntegerOverflow=off  RndMeth=Floor
  Rate Transition1 : RateTransition  OutPortSampleTime=qc_get_step_size*20
  Rate Transition2 : RateTransition  OutPortSampleTime=qc_get_step_size
  Stream Server : quarc_library/Communications/Basic/Stream Server  uri_source=Specify via dialog (evaluate)  uri=QD2CFG.uri_puente  send_buffer_size=1460  receive_buffer_size=1460  byte_order=little endian (Intel - LSB first)  optimization=Minimum latency  send_options=Send most recent data  receive_options=Receive most recent data  default_value=zeros(32,1)  sample_time=qc_get_step_size*20  active=off  implementation=Use blocking I/O in a separate thread  send_fifo_size=1000  receive_fifo_size=1000  send_priority=0  receive_priority=0  send_dimensions=off  receive_dimensions=off  max_dimensions=-1  data_type=double  type_expr=BusObject
      settings: AttributesFormatString="\"tcpip://localhost:18700\""
  Terminator1 : Terminator
  Terminator2 : Terminator
  Terminator3 : Terminator
  Python Commands [32] : Outport
  Python Connected (0,1) : Outport  Port=2
  wires:
  Telemetry [64]/1 -> Rate Transition1/1
  Rate Transition1/1 -> Stream Server/1
  Constant/1 -> Stream Server/2
  Stream Server/1 -> Connected/1
  Connected/1 -> Data Type Conversion/1
  Data Type Conversion/1 -> Python Connected (0,1)/1
  Stream Server/2 -> Terminator1/1
  Stream Server/3 -> Terminator2/1
  Stream Server/4 -> Rate Transition2/1
  Rate Transition2/1 -> Python Commands [32]/1
  Stream Server/5 -> Terminator3/1

== system QD2_MissionCtrl_Dual_MPC/Communication QDrone 1/Detect Communication loss ==
  note: Check if stream is 2 (connected) and error is positive (error codes are negative). Otherwise issue a communication error.
  State : Inport
  Error : Inport  Port=2
  Data Type Conversion : DataTypeConversion  SaturateOnIntegerOverflow=off  RndMeth=Floor
  MATLAB Function : MATLAB Function  TreatAsAtomicUnit=on
  Terminator2 : Terminator
  Threshold : quarc_library/Discontinuities/Threshold  operator=>=  param_src=Specify via dialog  threshold=0.5  duration=0.1
      settings: SourceProductName=QUARC Targets
  Time : quarc_library/Sources/Time/Time  time_source=Wall clock  sample_time=qc_get_step_size
  Communication Issue (0,1) : Outport  VectorParamsAs1DForOutWhenUnconnected=off
  wires:
  Error/1 -> MATLAB Function/3(error)
  MATLAB Function/1(stream_connection_loss) -> Threshold/1
  State/1 -> MATLAB Function/2(state)
  Time/1 -> MATLAB Function/1(time)
  Threshold/2 -> Terminator2/1
  Data Type Conversion/1 -> Communication Issue (0,1)/1
  Threshold/1 -> Data Type Conversion/1

== system QD2_MissionCtrl_Dual_MPC/Communication QDrone 2/Detect Communication loss ==
  note: Check if stream is 2 (connected) and error is positive (error codes are negative). Otherwise issue a communication error.
  State : Inport
  Error : Inport  Port=2
  Data Type Conversion : DataTypeConversion  SaturateOnIntegerOverflow=off  RndMeth=Floor
  MATLAB Function : MATLAB Function  TreatAsAtomicUnit=on
  Terminator2 : Terminator
  Threshold : quarc_library/Discontinuities/Threshold  operator=>=  param_src=Specify via dialog  threshold=0.5  duration=0.1
      settings: SourceProductName=QUARC Targets
  Time : quarc_library/Sources/Time/Time  time_source=Wall clock  sample_time=qc_get_step_size
  Communication Issue (0,1) : Outport  VectorParamsAs1DForOutWhenUnconnected=off
  wires:
  Threshold/1 -> Data Type Conversion/1
  Data Type Conversion/1 -> Communication Issue (0,1)/1
  Threshold/2 -> Terminator2/1
  Time/1 -> MATLAB Function/1(time)
  State/1 -> MATLAB Function/2(state)
  MATLAB Function/1(stream_connection_loss) -> Threshold/1
  Error/1 -> MATLAB Function/3(error)

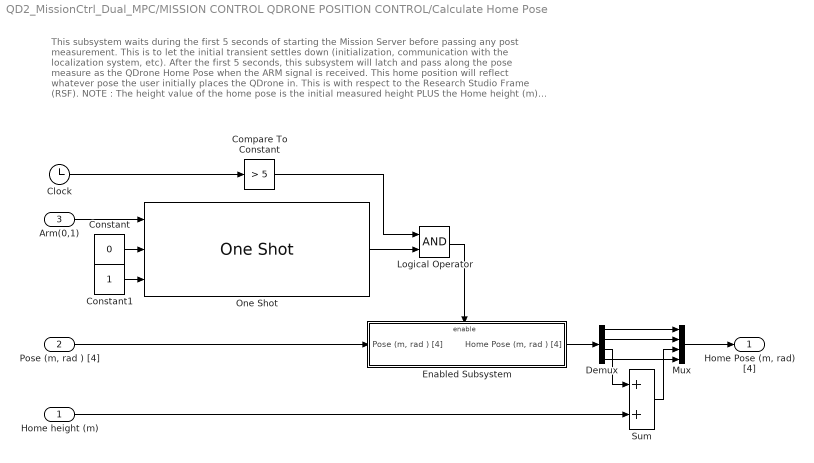
== system QD2_MissionCtrl_Dual_MPC/MISSION CONTROL QDRONE POSITION CONTROL/Calculate Home Pose ==
  note: This subsystem waits during the first 5 seconds of starting the Mission Server before passing any post measurement.
      | This is to let the initial transient settles down (initialization, communication with the localization system, etc).
      | After the first 5 seconds, this subsystem will latch and pass along the pose measure as the QDrone Home Pose when
      | the ARM signal is received.
      | This home position will reflect whatever pose the user initially places the QDrone in.
      | This is with respect to the Research Studio Frame (RSF).
      |
      | NOTE : The height value of the home pose is the initial measured height PLUS the Home height (m) input value.
  Home height (m) : Inport
  "Pose (m, rad ) [4]" : Inport  Port=2
  Arm(0,1) : Inport  Port=3
  Clock : Clock
  Compare To Constant : simulink/Logic and Bit Operations/Compare To Constant  relop=>  const=5  OutDataTypeStr=boolean
  Constant : Constant  Value=0
  Constant1 : Constant
  Demux : Demux
  Enabled Subsystem : Subsystem  TreatAsAtomicUnit=on
  Logical Operator : Logic  AllPortsSameDT=off  OutDataTypeStr=boolean
  Mux : Mux
  One Shot : quarc_library/Discontinuities/One Shot  trigger_type=Rising edge  redun_pulse=Ignore extraneous pulse  width_source=Specify via dialog  pulse_width=1/qc_get_step_size
      settings: SourceProductName=QUARC Targets
  Sum : Sum
  "Home Pose (m, rad) [4]" : Outport  VectorParamsAs1DForOutWhenUnconnected=off
  wires:
  Constant/1 -> One Shot/2
  Constant1/1 -> One Shot/3
  Arm(0,1)/1 -> One Shot/1
  One Shot/1 -> Logical Operator/2
  "Pose (m, rad ) [4]"/1 -> Enabled Subsystem/1("Pose (m, rad ) [4] ")
  Clock/1 -> Compare To Constant/1
  Compare To Constant/1 -> Logical Operator/1
  Logical Operator/1 -> Enabled Subsystem/Enable
  Enabled Subsystem/1("Home Pose (m, rad ) [4]") -> Demux/1
  Demux/1 -> Mux/1
  Demux/2 -> Mux/2
  Demux/4 -> Mux/4
  Demux/3 -> Sum/1
  Sum/1 -> Mux/3
  Home height (m)/1 -> Sum/2
  Mux/1 -> "Home Pose (m, rad) [4]"/1

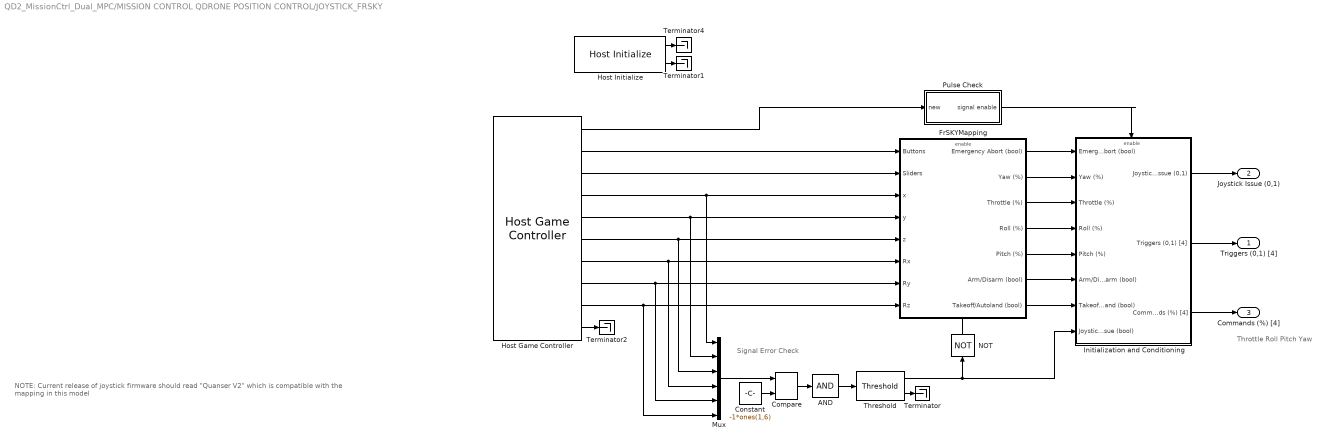
== system QD2_MissionCtrl_Dual_MPC/MISSION CONTROL QDRONE POSITION CONTROL/JOYSTICK_FRSKY ==
  note: Throttle
      | Roll
      | Pitch
      | Yaw
  note: Signal Error Check
  note: NOTE: Current release of joystick firmware should read "Quanser V2" which is compatible with the mapping in this model
  AND : Logic  Inputs=1  AllPortsSameDT=off  OutDataTypeStr=boolean
  Compare : quarc_library/Logic Operations/Compare  operator===  output_data_type=boolean
      settings: SourceProductName=QUARC Targets
  Constant : Constant  Value=-1*ones(1,6)
  FrSKYMapping : Subsystem
  Host Game Controller : quarc_library/Devices/Peripherals/Host/Host Game Controller  object_name=Host-1  controller=1  buffer_size=20  deadzone=[]  saturation=[]  sample_time=qc_get_step_size  auto_center=off  enabled=on  debug_mode=off
      settings: SourceProductName=QUARC Targets
  Host Initialize : quarc_library/Devices/Peripherals/Host/Host Initialize  object_name=Host-1  uri_source=Use external mode communications  uri=tcpip://localhost:18001  send_buffer_size=1000  receive_buffer_size=1000  thread_priority=0  run_client=on  use_window=off  window_position=[]  sample_time=qc_get_step_size  active=on
      settings: SourceProductName=QUARC Targets
  Initialization and Conditioning : Subsystem  TreatAsAtomicUnit=on
  Mux : Mux  Inputs=6
  NOT : Logic  Operator=NOT  IconShape=distinctive  AllPortsSameDT=off  OutDataTypeStr=boolean
  Pulse Check : Subsystem  TreatAsAtomicUnit=on
  Terminator{,1..2,4} (4 alike) : Terminator
  Threshold : quarc_library/Discontinuities/Threshold  operator=>=  param_src=Specify via dialog  threshold=0.5  duration=0.2
      settings: SourceProductName=QUARC Targets
  Triggers (0,1) [4] : Outport  VectorParamsAs1DForOutWhenUnconnected=off
  Joystick Issue (0,1) : Outport  Port=2  VectorParamsAs1DForOutWhenUnconnected=off
  Commands (%) [4] : Outport  Port=3  VectorParamsAs1DForOutWhenUnconnected=off
  wires:
  Host Game Controller/10 -> Terminator2/1
  Pulse Check/1(signal enable) -> Initialization and Conditioning/Enable
  Host Initialize/1 -> Terminator4/1
  FrSKYMapping/6("Arm/Disarm (bool) ") -> Initialization and Conditioning/6(Arm/Disarm (bool))
  Host Initialize/2 -> Terminator1/1
  FrSKYMapping/7(Takeoff/Autoland (bool)) -> Initialization and Conditioning/7(Takeoff/AutoLand (bool))
  Host Game Controller/7 -> Mux/4, FrSKYMapping/6(Rx)
  Host Game Controller/8 -> Mux/5, FrSKYMapping/7(Ry)
  Initialization and Conditioning/3(Commands (%) [4]) -> Commands (%) [4]/1
  Host Game Controller/5 -> Mux/2, FrSKYMapping/4(y)
  Host Game Controller/9 -> Mux/6, FrSKYMapping/8(Rz)
  Host Game Controller/1 -> Pulse Check/1(new)
  Mux/1 -> Compare/1
  Threshold/1 -> NOT/1, Initialization and Conditioning/8(Joystick Issue (bool))
  AND/1 -> Threshold/1
  Host Game Controller/3 -> FrSKYMapping/2(Sliders)
  Threshold/2 -> Terminator/1
  NOT/1 -> FrSKYMapping/Enable
  Constant/1 -> Compare/2
  Host Game Controller/6 -> Mux/3, FrSKYMapping/5(z)
  FrSKYMapping/4(Roll (%)) -> Initialization and Conditioning/4(Roll (%))
  FrSKYMapping/5(Pitch (%)) -> Initialization and Conditioning/5(Pitch (%))
  Compare/1 -> AND/1
  FrSKYMapping/1(Emergency Abort (bool)) -> Initialization and Conditioning/1(Emergency Abort (bool))
  Initialization and Conditioning/1(Joystick Issue (0,1)) -> Joystick Issue (0,1)/1
  Initialization and Conditioning/2(Triggers (0,1) [4]) -> Triggers (0,1) [4]/1
  FrSKYMapping/2(Yaw (%)) -> Initialization and Conditioning/2(Yaw (%))
  Host Game Controller/4 -> Mux/1, FrSKYMapping/3(x)
  Host Game Controller/2 -> FrSKYMapping/1(Buttons)
  FrSKYMapping/3(Throttle (%)) -> Initialization and Conditioning/3(Throttle (%))

== system QD2_MissionCtrl_Dual_MPC/MISSION CONTROL QDRONE POSITION CONTROL/Localization - Optitrack ==
  note: Double-click on the OptiTrack Trackables block.
      |
      | Click on the ... icon under Calibration file: and select the .cal file
      | created when calibrating the Optitrack cameras
      |
      | Click on the ... icon under Trackables definition file: and select
      | the trackables file created when defining rigid bodies (for the
      | QDrone you are about to use)
  For Each Subsystem (Convention Correction: Motive Frame to Research Studio Frame) : Subsystem  TreatAsAtomicUnit=on
  OptiTrack Trackables : quarc_library/Devices/Third-Party/NaturalPoint/OptiTrack/OptiTrack Trackables  calibration_file=C:\Users\user\Documents\OptiTrack\Nov 20_Team2\Calibration Exceptional (MeanErr 0.494 mm) 2026-11-20 7.cal  rigid_body_file=C:\Users\user\Documents\OptiTrack\Nov 20_Team2\RigidBody.motive  rigid_body_ids=QD2CFG.optitrack.rb_ids  sample_time=qc_get_step_size*10  active=off
      settings: SourceProductName=QUARC Targets
  Rate Transition1 : RateTransition
  Rate Transition2 : RateTransition
  Terminator1 : Terminator
  Terminator2 : Terminator
  Terminator3 : Terminator
  Data [7n] : Outport  VectorParamsAs1DForOutWhenUnconnected=off
  q [4n] : Outport  Port=2  VectorParamsAs1DForOutWhenUnconnected=off
  wires:
  OptiTrack Trackables/3 -> For Each Subsystem (Convention Correction: Motive Frame to Research Studio Frame)/3(rot_MF (rad) [3n])
  OptiTrack Trackables/2 -> For Each Subsystem (Convention Correction: Motive Frame to Research Studio Frame)/2(q_MF [4n])
  OptiTrack Trackables/1 -> For Each Subsystem (Convention Correction: Motive Frame to Research Studio Frame)/1(xyz_MF (m) [3n])
  Rate Transition2/1 -> Data [7n]/1
  OptiTrack Trackables/4 -> For Each Subsystem (Convention Correction: Motive Frame to Research Studio Frame)/4(isTracking [n])
  For Each Subsystem (Convention Correction: Motive Frame to Research Studio Frame)/5("data_RSF (m, rad, bool) [7n]") -> Rate Transition2/1
  For Each Subsystem (Convention Correction: Motive Frame to Research Studio Frame)/2(xyz_RSF (m) [3n]) -> Terminator1/1
  For Each Subsystem (Convention Correction: Motive Frame to Research Studio Frame)/3(rot_RSF (rad) [3n]) -> Terminator2/1
  For Each Subsystem (Convention Correction: Motive Frame to Research Studio Frame)/4(isTracking_RSF [n]) -> Terminator3/1
  For Each Subsystem (Convention Correction: Motive Frame to Research Studio Frame)/1(q_RSF [4n]) -> Rate Transition1/1
  Rate Transition1/1 -> q [4n]/1
